simulink subsystem "matlab_mission_manager"  (R2026a)
settings: Solver=VariableStepAuto
undefined symbols (not defined in the file): S
PreSaveFcn:
  | defaultToFileBlockNames(bdroot);
settings Model: Creator=kjhaydon  LastModifiedBy=kjhaydon

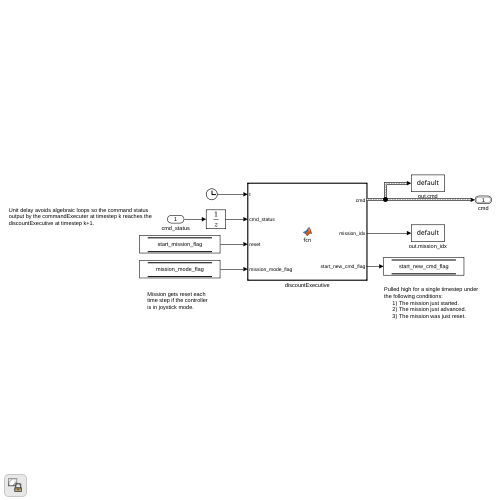
[thumbnail: Simulink's stored preview of the top-level diagram]
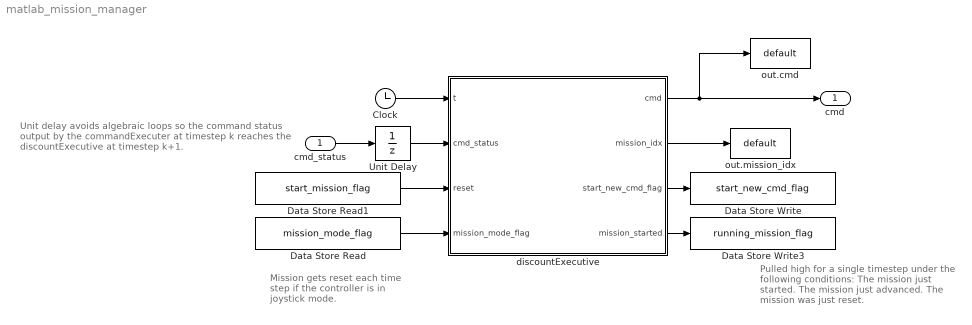
== system matlab_mission_manager ==
  note: Pulled high for a single timestep under the following conditions:
      | The mission just started.
      | The mission just advanced.
      | The mission was just reset.
  note: Unit delay avoids algebraic loops so the command status
      | output by the commandExecuter at timestep k reaches the
      | discountExecutive at timestep k+1.
  note: Mission gets reset each time step if the controller is in joystick mode.
  cmd_status : Inport  SampleTime=S.dt_control
  Clock : Clock
  Data Store Read : DataStoreRead  DataStoreName=mission_mode_flag  IndexOptions=Index vector (dialog)  Indices=1  OutputSizes=1
  Data Store Read1 : DataStoreRead  DataStoreName=start_mission_flag  IndexOptions=Index vector (dialog)  Indices=1  OutputSizes=1
  Data Store Write : DataStoreWrite  DataStoreName=start_new_cmd_flag  IndexOptions=Index vector (dialog)  Indices=1  OutputSizes=1
  Data Store Write3 : DataStoreWrite  DataStoreName=running_mission_flag  IndexOptions=Index vector (dialog)  Indices=1  OutputSizes=1
  Unit Delay : UnitDelay  InitialCondition=int8('RUNN')'  SampleTime=-1
  discountExecutive : MATLAB Function  TreatAsAtomicUnit=on
  out.cmd : ToFile  Filename=default  MatrixName=cmd  SaveFormat=Timeseries
  out.mission_idx : ToFile  Filename=default  MatrixName=mission_idx  SaveFormat=Timeseries
  cmd : Outport  OutDataTypeStr=Bus: cmd_bus
      settings: VarSizeSig=Yes
  wires:
  cmd_status/1 -> Unit Delay/1
  Data Store Read1/1 -> discountExecutive/3(reset)
  Unit Delay/1 -> discountExecutive/2(cmd_status)
  discountExecutive/2(mission_idx) -> out.mission_idx/1
  discountExecutive/1(cmd) -> out.cmd/1, cmd/1
  discountExecutive/3(start_new_cmd_flag) -> Data Store Write/1
  Clock/1 -> discountExecutive/1(t)
  Data Store Read/1 -> discountExecutive/4(mission_mode_flag)
  discountExecutive/4(mission_started) -> Data Store Write3/1

== matlab function matlab_mission_manager/discountExecutive ==
  settings: updateMethod=DISCRETE  sampleTime=S.dt_control
  data: t input; cmd_status input; cmd output Bus: cmd_bus; mission parameter Bus: cmd_bus size=max_commands_in_mission; mission_idx output; reset input boolean; start_new_cmd_flag output; mission_mode_flag input; mission_started output
function [cmd, mission_idx, start_new_cmd_flag, mission_started] = fcn(t, cmd_status, mission, reset, mission_mode_flag)

[cmd, mission_idx, start_new_cmd_flag, mission_started] = discountExecutive(t, cmd_status, mission, reset, mission_mode_flag);
